simulink model "ahm_model_no_actuators_AHS"  (R2024b)
settings: Solver=FixedStepAuto  StartTime=0.0  StopTime=TMax  FixedStep=dt  RelTol=1e-3
settings Model: Creator=mcdevin  LastModifiedBy=Andreas

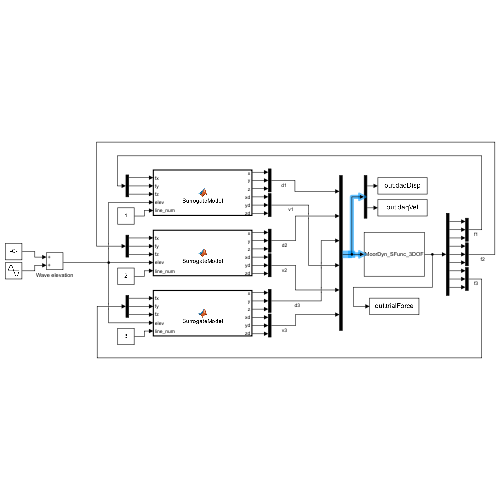
[thumbnail: Simulink's stored preview of the top-level diagram]
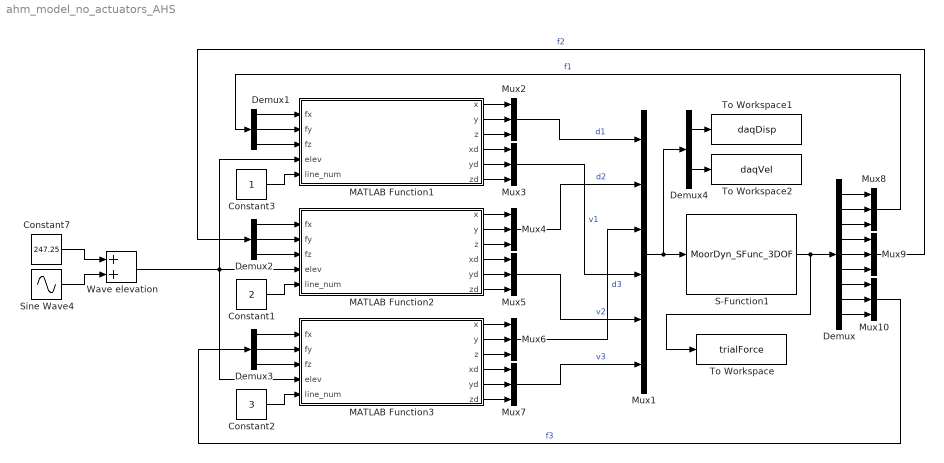
== system ahm_model_no_actuators_AHS ==
  Constant1 : Constant  Value=2
  Constant2 : Constant  Value=3
  Constant3 : Constant
  Constant7 : Constant  Value=247.25
  Demux : Demux  Outputs=9
  Demux1 : Demux  Outputs=3
  Demux2 : Demux  Outputs=3
  Demux3 : Demux  Outputs=3
  Demux4 : Demux  Outputs=[9 9]
  MATLAB Function1 : MATLAB Function  TreatAsAtomicUnit=on
  MATLAB Function2 : MATLAB Function  TreatAsAtomicUnit=on
  MATLAB Function3 : MATLAB Function  TreatAsAtomicUnit=on
  Mux1 : Mux  Inputs=6
  Mux{2..10} (9 alike) : Mux  Inputs=3
  S-Function1 : S-Function  FunctionName=MoorDyn_SFunc_3DOF  Parameters=MD_InputFileName, dt, TMax  SFunctionDeploymentMode=off  EnableBusSupport=off
  Sine Wave4 : Sin  Amplitude=0.5  Frequency=0.7330386  SampleTime=0
  To Workspace : ToWorkspace  VariableName=trialForce  SaveFormat=Timeseries  SampleTime=-1
  To Workspace1 : ToWorkspace  VariableName=daqDisp  SaveFormat=Timeseries  SampleTime=-1
  To Workspace2 : ToWorkspace  VariableName=daqVel  SaveFormat=Timeseries  SampleTime=-1
  Wave elevation : Sum
  wires:
  Constant3/1 -> MATLAB Function1/5(line_num)
  Sine Wave4/1 -> Wave elevation/2
  Constant7/1 -> Wave elevation/1
  Mux1/1 -> Demux4/1, S-Function1/1
  Constant1/1 -> MATLAB Function2/5(line_num)
  Wave elevation/1 -> MATLAB Function1/4(elev), MATLAB Function2/4(elev), MATLAB Function3/4(elev)
  Constant2/1 -> MATLAB Function3/5(line_num)
  MATLAB Function1/1(x) -> Mux2/1
  MATLAB Function1/2(y) -> Mux2/2
  MATLAB Function1/3(z) -> Mux2/3
  MATLAB Function1/4(xd) -> Mux3/1
  MATLAB Function1/5(yd) -> Mux3/2
  MATLAB Function1/6(zd) -> Mux3/3
  MATLAB Function3/1(x) -> Mux6/1
  MATLAB Function3/2(y) -> Mux6/2
  MATLAB Function3/3(z) -> Mux6/3
  MATLAB Function3/4(xd) -> Mux7/1
  MATLAB Function3/5(yd) -> Mux7/2
  MATLAB Function3/6(zd) -> Mux7/3
  MATLAB Function2/1(x) -> Mux4/1
  MATLAB Function2/2(y) -> Mux4/2
  MATLAB Function2/3(z) -> Mux4/3
  MATLAB Function2/4(xd) -> Mux5/1
  MATLAB Function2/5(yd) -> Mux5/2
  MATLAB Function2/6(zd) -> Mux5/3
  Mux2/1 -> Mux1/1  "d1"
  Mux4/1 -> Mux1/2  "d2"
  Mux6/1 -> Mux1/3  "d3"
  Mux3/1 -> Mux1/4  "v1"
  Mux5/1 -> Mux1/5  "v2"
  Mux7/1 -> Mux1/6  "v3"
  S-Function1/1 -> To Workspace/1, Demux/1
  Demux/1 -> Mux8/1
  Demux/2 -> Mux8/2
  Demux/3 -> Mux8/3
  Demux/4 -> Mux9/1
  Demux/5 -> Mux9/2
  Demux/6 -> Mux9/3
  Demux/7 -> Mux10/1
  Demux/8 -> Mux10/2
  Demux/9 -> Mux10/3
  Demux1/1 -> MATLAB Function1/1(fx)
  Demux1/2 -> MATLAB Function1/2(fy)
  Demux1/3 -> MATLAB Function1/3(fz)
  Demux2/1 -> MATLAB Function2/1(fx)
  Demux2/2 -> MATLAB Function2/2(fy)
  Demux2/3 -> MATLAB Function2/3(fz)
  Demux3/1 -> MATLAB Function3/1(fx)
  Demux3/2 -> MATLAB Function3/2(fy)
  Demux3/3 -> MATLAB Function3/3(fz)
  Mux8/1 -> Demux1/1  "f1"
  Mux9/1 -> Demux2/1  "f2"
  Mux10/1 -> Demux3/1  "f3"
  Demux4/1 -> To Workspace1/1
  Demux4/2 -> To Workspace2/1

== matlab function ahm_model_no_actuators_AHS/MATLAB Function1 ==
  data: fx input; x output; fy input; fz input; elev input; line_num input; y output; z output; xd output; yd output; zd output
function [x, y, z, xd, yd, zd]  = SurrogateModel(fx, fy, fz, elev, line_num)
    
    % preallocate outputs
    x = double(0);
    y = double(0);
    z = double(0);
    xd = double(0);
    yd = double(0);
    zd = double(0);

    % declare python functions and inputs
    coder.extrinsic('py.list')
    coder.extrinsic('py.predict_motions.predict_motions');
    inputs = py.list({fx, fy, fz, elev});

    % set surrogate model files
    switch(line_num)
        case 1
            model_x = 'models/model_l1px.h5';
            model_y = 'models/model_l1py.h5';
            model_z = 'models/model_l1pz.h5';
            model_xd = 'models/model_l1vx.h5';
            model_yd = 'models/model_l1vy.h5';
            model_zd = 'models/model_l1vz.h5';
        case 2
            model_x = 'models/model_l2px.h5';
            model_y = 'models/model_l2py.h5';
            model_z = 'models/model_l2pz.h5';
            model_xd = 'models/model_l2vx.h5';
            model_yd = 'models/model_l2vy.h5';
            model_zd = 'models/model_l2vz.h5';
        case 3
            model_x = 'models/model_l3px.h5';
            model_y = 'models/model_l3py.h5';
            model_z = 'models/model_l3pz.h5';
            model_xd = 'models/model_l3vx.h5';
            model_yd = 'models/model_l3vy.h5';
            model_zd = 'models/model_l3vz.h5';
        otherwise
            error('Invalid line number.');
    end
    
    % call surrogate model to predict positions and velocities
    x_py = py.predict_motions.predict_motions(model_x, inputs);
    y_py = py.predict_motions.predict_motions(model_y, inputs);
    z_py = py.predict_motions.predict_motions(model_z, inputs);
    xd_py = py.predict_motions.predict_motions(model_xd, inputs);
    yd_py = py.predict_motions.predict_motions(model_yd, inputs);
    zd_py = py.predict_motions.predict_motions(model_zd, inputs);

    % convert Python outputs to MATLAB data types
    x = double(x_py);
    y = double(y_py);
    z = double(z_py);
    xd = double(xd_py);
    yd = double(yd_py);
    zd = double(zd_py);
    
end

== matlab function ahm_model_no_actuators_AHS/MATLAB Function2 ==
  data: fx input; x output; fy input; fz input; elev input; line_num input; y output; z output; xd output; yd output; zd output
function [x, y, z, xd, yd, zd]  = SurrogateModel(fx, fy, fz, elev, line_num)
    
    % preallocate outputs
    x = double(0);
    y = double(0);
    z = double(0);
    xd = double(0);
    yd = double(0);
    zd = double(0);

    % declare python functions and inputs
    coder.extrinsic('py.list')
    coder.extrinsic('py.predict_motions.predict_motions');
    inputs = py.list({fx, fy, fz, elev});

    % set surrogate model files
    switch(line_num)
        case 1
            model_x = 'models/model_l1px.h5';
            model_y = 'models/model_l1py.h5';
            model_z = 'models/model_l1pz.h5';
            model_xd = 'models/model_l1vx.h5';
            model_yd = 'models/model_l1vy.h5';
            model_zd = 'models/model_l1vz.h5';
        case 2
            model_x = 'models/model_l2px.h5';
            model_y = 'models/model_l2py.h5';
            model_z = 'models/model_l2pz.h5';
            model_xd = 'models/model_l2vx.h5';
            model_yd = 'models/model_l2vy.h5';
            model_zd = 'models/model_l2vz.h5';
        case 3
            model_x = 'models/model_l3px.h5';
            model_y = 'models/model_l3py.h5';
            model_z = 'models/model_l3pz.h5';
            model_xd = 'models/model_l3vx.h5';
            model_yd = 'models/model_l3vy.h5';
            model_zd = 'models/model_l3vz.h5';
        otherwise
            error('Invalid line number.');
    end
    
    % call surrogate model to predict positions and velocities
    x_py = py.predict_motions.predict_motions(model_x, inputs);
    y_py = py.predict_motions.predict_motions(model_y, inputs);
    z_py = py.predict_motions.predict_motions(model_z, inputs);
    xd_py = py.predict_motions.predict_motions(model_xd, inputs);
    yd_py = py.predict_motions.predict_motions(model_yd, inputs);
    zd_py = py.predict_motions.predict_motions(model_zd, inputs);

    % convert Python outputs to MATLAB data types
    x = double(x_py);
    y = double(y_py);
    z = double(z_py);
    xd = double(xd_py);
    yd = double(yd_py);
    zd = double(zd_py);

    
    
end

== matlab function ahm_model_no_actuators_AHS/MATLAB Function3 ==
  data: fx input; x output; fy input; fz input; elev input; line_num input; y output; z output; xd output; yd output; zd output
function [x, y, z, xd, yd, zd]  = SurrogateModel(fx, fy, fz, elev, line_num)
    
    % preallocate outputs
    x = double(0);
    y = double(0);
    z = double(0);
    xd = double(0);
    yd = double(0);
    zd = double(0);

    % declare python functions and inputs
    coder.extrinsic('py.list')
    coder.extrinsic('py.predict_motions.predict_motions');
    inputs = py.list({fx, fy, fz, elev});

    % set surrogate model files
    switch(line_num)
        case 1
            model_x = 'models/model_l1px.h5';
            model_y = 'models/model_l1py.h5';
            model_z = 'models/model_l1pz.h5';
            model_xd = 'models/model_l1vx.h5';
            model_yd = 'models/model_l1vy.h5';
            model_zd = 'models/model_l1vz.h5';
        case 2
            model_x = 'models/model_l2px.h5';
            model_y = 'models/model_l2py.h5';
            model_z = 'models/model_l2pz.h5';
            model_xd = 'models/model_l2vx.h5';
            model_yd = 'models/model_l2vy.h5';
            model_zd = 'models/model_l2vz.h5';
        case 3
            model_x = 'models/model_l3px.h5';
            model_y = 'models/model_l3py.h5';
            model_z = 'models/model_l3pz.h5';
            model_xd = 'models/model_l3vx.h5';
            model_yd = 'models/model_l3vy.h5';
            model_zd = 'models/model_l3vz.h5';
        otherwise
            error('Invalid line number.');
    end
    
    % call surrogate model to predict positions and velocities
    x_py = py.predict_motions.predict_motions(model_x, inputs);
    y_py = py.predict_motions.predict_motions(model_y, inputs);
    z_py = py.predict_motions.predict_motions(model_z, inputs);
    xd_py = py.predict_motions.predict_motions(model_xd, inputs);
    yd_py = py.predict_motions.predict_motions(model_yd, inputs);
    zd_py = py.predict_motions.predict_motions(model_zd, inputs);

    % convert Python outputs to MATLAB data types
    x = double(x_py);
    y = double(y_py);
    z = double(z_py);
    xd = double(xd_py);
    yd = double(yd_py);
    zd = double(zd_py);

end
